simulink model "exp_001_buckopenloop"  (R2025b)
settings: Solver=VariableStepAuto  StartTime=0.0  StopTime=0.2  RelTol=1e-5
model workspace (MAT data in the model file):
  Vin = 155
undefined symbols (not defined in the file): Cout, D0, L, Rload, Tsoft
libraries: simulink x1
settings Model: Creator=qq  LastModifiedBy=qq

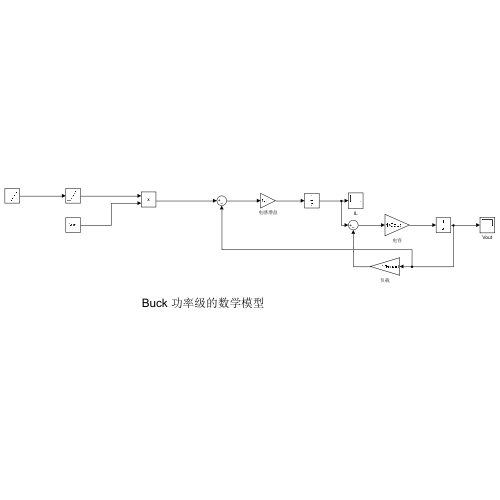
[thumbnail: Simulink's stored preview of the top-level diagram]
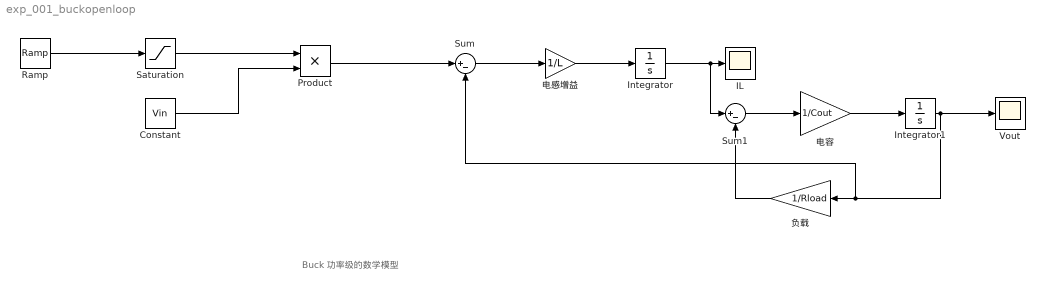
== system exp_001_buckopenloop ==
  note: Buck 功率级的数学模型
  Constant : Constant  Value=Vin
  IL : Scope
      settings: ActiveDisplayYMinimum=0.54418009313796034  ActiveDisplayYMaximum=20.620576330847424
  Integrator : Integrator
  Integrator1 : Integrator
  Product : Product
  Ramp : simulink/Sources/Ramp  slope=D0/Tsoft  start=0  InitialOutput=0
  Saturation : Saturate  UpperLimit=D0  LowerLimit=0
  Sum : Sum  Inputs=|+-
  Sum1 : Sum  Inputs=|+-
  Vout : Scope
      settings: ActiveDisplayYMinimum=-12.634597329928301  ActiveDisplayYMaximum=113.71137596935475
  电容 : Gain  Gain=1/Cout
  电感增益 : Gain  Gain=1/L
  负载 : Gain  Gain=1/Rload
  wires:
  Ramp/1 -> Saturation/1
  Saturation/1 -> Product/1
  Constant/1 -> Product/2
  Product/1 -> Sum/1
  Sum/1 -> 电感增益/1
  Integrator/1 -> Sum1/1, IL/1
  电感增益/1 -> Integrator/1
  Sum1/1 -> 电容/1
  电容/1 -> Integrator1/1
  Integrator1/1 -> 负载/1, Sum/2, Vout/1
  负载/1 -> Sum1/2
